simulink model "PI_controller"  (R2026a)
settings: Solver=VariableStepAuto  StopTime=2
values from neighbouring files (symbols this model uses):
  D = 0.0000188    (= 1.88e-05)    [measurements.m]    (also in motor_model_m.m = 5e-05; run_simulink.m = 5e-05; run_simulink_PI_Controller.m = 5e-05; run_simulink_turnrate_Controller.m = 5e-05)
  J = -b / a    (= 2.25042607204e-06)    [measurements.m]    (also in motor_model_m.m = 5.56231644013e-06; run_simulink.m = 5.56231644013e-06; run_simulink_PI_Controller.m = 5.56231644013e-06; run_simulink_turnrate_Controller.m = 5.56231644013e-06)
  Kb = Kt    (= 0.009)    [motor_model_m.m]    (also in run_simulink.m; run_simulink_PI_Controller.m; run_simulink_turnrate_Controller.m; run_simulink_turnrate_Controller_Heading.m)
  Kp = 0.1202    [motor_model_m.m]    (also in run_simulink.m; run_simulink_PI_Controller.m; run_simulink_turnrate_Controller.m; run_simulink_turnrate_Controller_Heading.m)
  Kt = 0.009    [motor_model_m.m]    (also in run_simulink.m; run_simulink_PI_Controller.m; run_simulink_turnrate_Controller.m; run_simulink_turnrate_Controller_Heading.m)
  L = 5.15e-3    (= 0.00515)    [measurements.m]    (also in motor_model_m.m = 0.0045; run_simulink.m = 0.0045; run_simulink_PI_Controller.m = 0.0045; run_simulink_turnrate_Controller.m = 0.0045)
  R = 4.29    [measurements.m]    (also in motor_model_m.m; run_simulink.m; run_simulink_PI_Controller.m; run_simulink_turnrate_Controller.m)
  r2m = wheelRadius/gear    (= 0.00309917355372)    [motor_model_m.m]    (also in run_simulink.m; run_simulink_PI_Controller.m; run_simulink_turnrate_Controller.m; run_simulink_turnrate_Controller_Heading.m)
  Ti = 0.0685    [motor_model_m.m]    (also in run_simulink_PI_Controller.m; run_simulink_turnrate_Controller.m; run_simulink_turnrate_Controller_Heading.m)
settings Model: Creator=chr  LastModifiedBy=luma

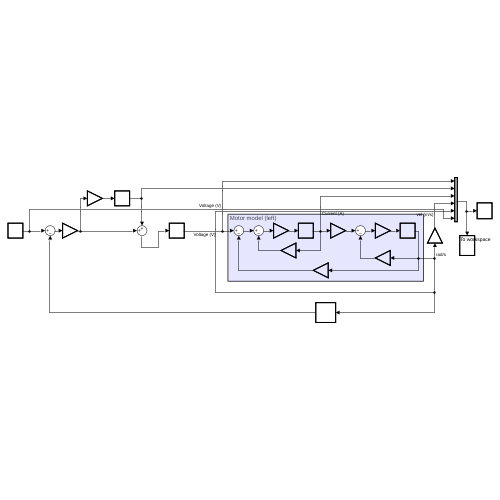
[thumbnail: Simulink's stored preview of the top-level diagram]
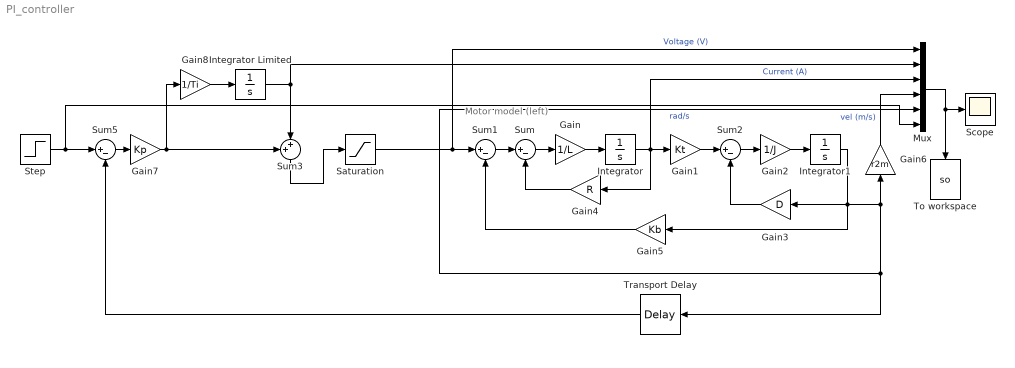
== system PI_controller ==
  note: Motor model (left)
  Gain : Gain  Gain=1/L
  Gain1 : Gain  Gain=Kt
  Gain2 : Gain  Gain=1/J
  Gain3 : Gain  Gain=D
  Gain4 : Gain  Gain=R
  Gain5 : Gain  Gain=Kb
  Gain6 : Gain  Gain=r2m
  Gain7 : Gain  Gain=Kp
  Gain8 : Gain  Gain=1/Ti
  Integrator : Integrator
  Integrator Limited : Integrator  LimitOutput=on  UpperSaturationLimit=8  LowerSaturationLimit=-8
  Integrator1 : Integrator
  Mux : Mux  Inputs=6
  Saturation : Saturate  UpperLimit=8  LowerLimit=-8
  Scope : Scope
      settings: ActiveDisplayYMinimum=-3.3889972018890928  ActiveDisplayYMaximum=6.5603329891550111
  Step : Step  Time=0.1  FinalValue=100  SampleTime=0
  Sum{,1..2,5} (4 alike) : Sum  Inputs=|+-
  Sum3 : Sum  Inputs=++|
  To workspace : ToWorkspace  VariableName=so  SampleTime=-1
      settings: Save2DSignal=2-D array (concatenate along first dimension)
  Transport Delay : TransportDelay  DelayTime=0.01
  wires:
  Gain/1 -> Integrator/1
  Sum/1 -> Gain/1
  Integrator/1 -> Mux/3, Gain4/1, Gain1/1  "Current (A)"
  Sum1/1 -> Sum/1
  Gain1/1 -> Sum2/1
  Sum2/1 -> Gain2/1
  Gain2/1 -> Integrator1/1
  Integrator1/1 -> Gain3/1, Gain5/1, Transport Delay/1, Mux/5, Gain6/1  "rad/s"
  Gain3/1 -> Sum2/2
  Gain4/1 -> Sum/2
  Gain5/1 -> Sum1/2
  Mux/1 -> Scope/1, To workspace/1
  Gain6/1 -> Mux/4  "vel (m/s)"
  Saturation/1 -> Mux/1, Sum1/1  "Voltage (V)"
  Step/1 -> Mux/6, Sum5/1
  Transport Delay/1 -> Sum5/2
  Sum5/1 -> Gain7/1
  Gain7/1 -> Gain8/1, Sum3/1
  Gain8/1 -> Integrator Limited/1
  Integrator Limited/1 -> Mux/2, Sum3/2
  Sum3/1 -> Saturation/1
